simulink model "SensorlessHandover"  (R2026b)
settings: Solver=VariableStepAuto
undefined symbols (not defined in the file or in its folder): fusionCfg, handoverCfg
settings Model: Creator=24322  LastModifiedBy=24322

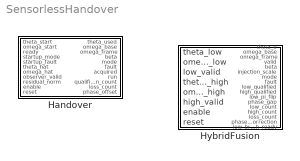
== system SensorlessHandover ==
  Handover : Subsystem  mask{handoverCfg=handoverCfg}
      mask prompts: handoverCfg "Handover configuration"
  HybridFusion : Subsystem  mask{fusionCfg=fusionCfg}
      mask prompts: fusionCfg "Two-tracker fusion configuration"

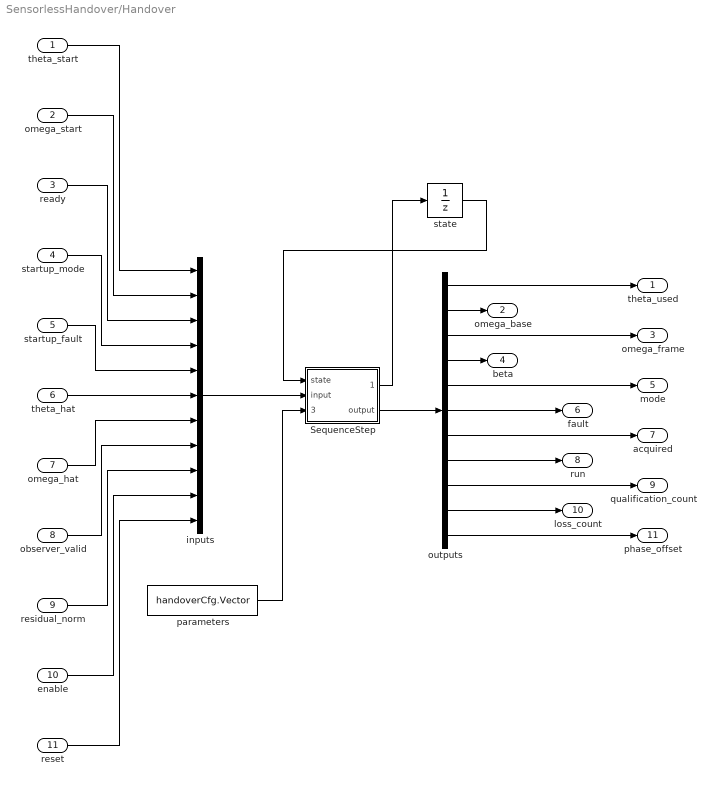
== system SensorlessHandover/Handover ==
  theta_start : Inport  SampleTime=handoverCfg.Ts
  omega_start : Inport  Port=2  SampleTime=handoverCfg.Ts
  ready : Inport  Port=3  SampleTime=handoverCfg.Ts
  startup_mode : Inport  Port=4  SampleTime=handoverCfg.Ts
  startup_fault : Inport  Port=5  SampleTime=handoverCfg.Ts
  theta_hat : Inport  Port=6  SampleTime=handoverCfg.Ts
  omega_hat : Inport  Port=7  SampleTime=handoverCfg.Ts
  observer_valid : Inport  Port=8  SampleTime=handoverCfg.Ts
  residual_norm : Inport  Port=9  SampleTime=handoverCfg.Ts
  enable : Inport  Port=10  SampleTime=handoverCfg.Ts
  reset : Inport  Port=11  SampleTime=handoverCfg.Ts
  SequenceStep : MATLAB Function  TreatAsAtomicUnit=on
  inputs : Mux  Inputs=11
  outputs : Demux  Outputs=11
  parameters : Constant  Value=handoverCfg.Vector
  state : UnitDelay  InitialCondition=handoverCfg.State0  SampleTime=handoverCfg.Ts
  theta_used : Outport
  omega_base : Outport  Port=2
  omega_frame : Outport  Port=3
  beta : Outport  Port=4
  mode : Outport  Port=5
  fault : Outport  Port=6
  acquired : Outport  Port=7
  run : Outport  Port=8
  qualification_count : Outport  Port=9
  loss_count : Outport  Port=10
  phase_offset : Outport  Port=11
  wires:
  outputs/11 -> phase_offset/1
  outputs/10 -> loss_count/1
  outputs/9 -> qualification_count/1
  outputs/8 -> run/1
  outputs/7 -> acquired/1
  outputs/6 -> fault/1
  outputs/5 -> mode/1
  outputs/4 -> beta/1
  outputs/3 -> omega_frame/1
  outputs/2 -> omega_base/1
  outputs/1 -> theta_used/1
  reset/1 -> inputs/11
  enable/1 -> inputs/10
  residual_norm/1 -> inputs/9
  observer_valid/1 -> inputs/8
  omega_hat/1 -> inputs/7
  theta_hat/1 -> inputs/6
  startup_fault/1 -> inputs/5
  startup_mode/1 -> inputs/4
  ready/1 -> inputs/3
  omega_start/1 -> inputs/2
  theta_start/1 -> inputs/1
  SequenceStep/2(output) -> outputs/1
  SequenceStep/1(nextState) -> state/1
  parameters/1 -> SequenceStep/3(parameter)
  inputs/1 -> SequenceStep/2(input)
  state/1 -> SequenceStep/1(state)

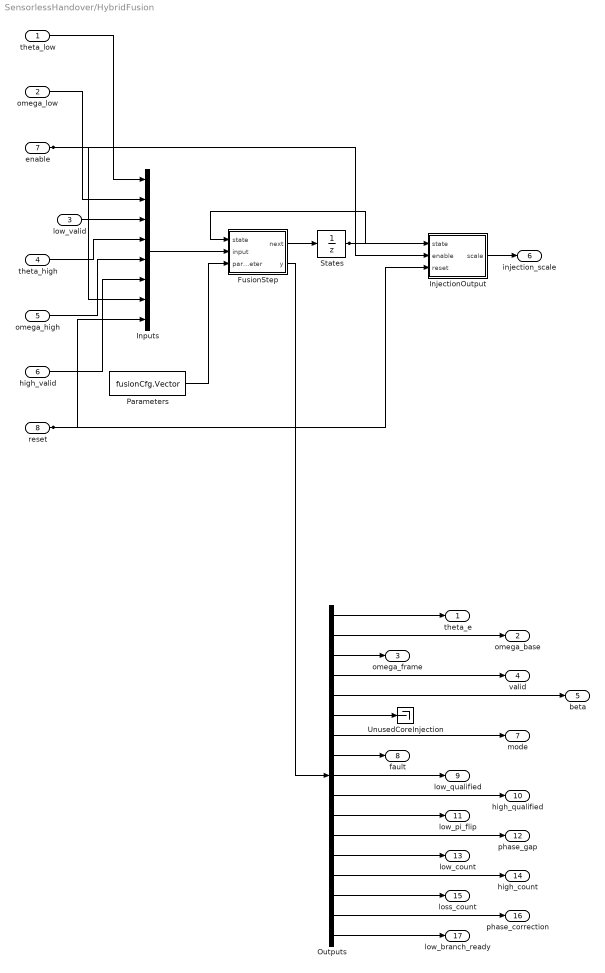
== system SensorlessHandover/HybridFusion ==
  theta_low : Inport  SampleTime=fusionCfg.Ts
  omega_low : Inport  Port=2  SampleTime=fusionCfg.Ts
  low_valid : Inport  Port=3  SampleTime=fusionCfg.Ts
  theta_high : Inport  Port=4  SampleTime=fusionCfg.Ts
  omega_high : Inport  Port=5  SampleTime=fusionCfg.Ts
  high_valid : Inport  Port=6  SampleTime=fusionCfg.Ts
  enable : Inport  Port=7  SampleTime=fusionCfg.Ts
  reset : Inport  Port=8  SampleTime=fusionCfg.Ts
  FusionStep : MATLAB Function  TreatAsAtomicUnit=on
  InjectionOutput : MATLAB Function  TreatAsAtomicUnit=on
  Inputs : Mux  Inputs=8
  Outputs : Demux  Outputs=17
  Parameters : Constant  Value=fusionCfg.Vector
  States : UnitDelay  InitialCondition=fusionCfg.State0  SampleTime=fusionCfg.Ts
  UnusedCoreInjection : Terminator
  theta_e : Outport
  omega_base : Outport  Port=2
  omega_frame : Outport  Port=3
  valid : Outport  Port=4
  beta : Outport  Port=5
  injection_scale : Outport  Port=6
  mode : Outport  Port=7
  fault : Outport  Port=8
  low_qualified : Outport  Port=9
  high_qualified : Outport  Port=10
  low_pi_flip : Outport  Port=11
  phase_gap : Outport  Port=12
  low_count : Outport  Port=13
  high_count : Outport  Port=14
  loss_count : Outport  Port=15
  phase_correction : Outport  Port=16
  low_branch_ready : Outport  Port=17
  wires:
  Outputs/17 -> low_branch_ready/1
  Outputs/16 -> phase_correction/1
  Outputs/15 -> loss_count/1
  Outputs/14 -> high_count/1
  Outputs/13 -> low_count/1
  Outputs/12 -> phase_gap/1
  Outputs/11 -> low_pi_flip/1
  Outputs/10 -> high_qualified/1
  Outputs/9 -> low_qualified/1
  Outputs/8 -> fault/1
  Outputs/7 -> mode/1
  InjectionOutput/1(scale) -> injection_scale/1
  Outputs/5 -> beta/1
  Outputs/4 -> valid/1
  Outputs/3 -> omega_frame/1
  Outputs/2 -> omega_base/1
  Outputs/1 -> theta_e/1
  reset/1 -> InjectionOutput/3(reset), Inputs/8
  enable/1 -> Inputs/7, InjectionOutput/2(enable)
  high_valid/1 -> Inputs/6
  omega_high/1 -> Inputs/5
  theta_high/1 -> Inputs/4
  low_valid/1 -> Inputs/3
  omega_low/1 -> Inputs/2
  theta_low/1 -> Inputs/1
  Outputs/6 -> UnusedCoreInjection/1
  FusionStep/2(y) -> Outputs/1
  FusionStep/1(next) -> States/1
  Parameters/1 -> FusionStep/3(parameter)
  Inputs/1 -> FusionStep/2(input)
  States/1 -> FusionStep/1(state), InjectionOutput/1(state)

== matlab function SensorlessHandover/HybridFusion/FusionStep ==
  data: next output; state input; y output; input input; parameter input
function [next,y]=hybrid_fusion_step(state,input,parameter)
%HYBRID_FUSION_STEP Qualified bidirectional fusion; no motor truth inputs.
% input: thetaLow,omegaLow,lowValid,thetaHigh,omegaHigh,highValid,enable,reset.
% y: theta,omegaBase,omegaFrame,valid,beta,injection,mode,fault,lowQ,highQ,
%    lowPiFlip,phaseGap,lowN,highN,lossN,phaseCorrection,lowBranchReady.
% Modes: 0 wait,1 low,2 blend,3 high,4 latched fault.
%#codegen
p=cast(parameter,'like',state);u=cast(input,'like',state);
next=state;y=zeros(17,1,'like',state);
if ~isfinite(u(7)) || ~isfinite(u(8))
    next(10)=2;next(4)=0;y(1)=state(1);y(7)=4;y(8)=2;return
end
if u(7)<.5 || u(8)>.5
    next(:)=0;next(4)=1;next(18)=1;return
end
if state(10)>0
    next(4)=0;y(1)=state(1);y(7)=4;y(8)=state(10);return
end

rawLow=all(isfinite(u(1:3))) && u(3)>.5 && abs(u(2))<=p(4) && state(4)>=p(17);
rawHigh=all(isfinite(u(4:6))) && u(6)>.5 && abs(u(5))>=p(16);
if rawLow && state(15)>.5
    rawLow=abs(wrap(u(1)-state(11)-p(1)*state(12)))<=p(14);
end
if rawHigh && state(16)>.5
    rawHigh=abs(wrap(u(4)-state(13)-p(1)*state(14)))<=p(14);
end
if rawLow
    next(11)=u(1);next(12)=u(2);next(15)=1;
elseif state(15)>.5
    next(11)=wrap(state(11)+p(1)*state(12));
end
if rawHigh
    next(13)=u(4);next(14)=u(5);next(16)=1;
elseif state(16)>.5
    next(13)=wrap(state(13)+p(1)*state(14));
end

flip=state(5);branch=state(17);gap=cast(0,'like',state);
if state(4)<p(17),branch=cast(0,'like',state);end
highWasQualified=state(7)>=p(7) && rawHigh;
if state(9)>.5 && state(3)>=1 && highWasQualified && rawLow && (branch<.5 || state(6)<1)
    ordinary=abs(wrap(u(1)-u(4)));opposite=abs(wrap(u(1)+pi-u(4)));
    candidate=cast(opposite<ordinary,'like',state);
    candidateGap=wrap(u(4)-u(1)-pi*candidate);
    if abs(candidateGap)<=p(5) && abs(u(2)-u(5))<=p(6)
        flip=candidate;branch=cast(1,'like',state);
    else
        branch=cast(0,'like',state);
    end
end
thetaLow=cast(0,'like',state);
if rawLow,thetaLow=wrap(u(1)+pi*flip);end
agree=false;
if rawLow && rawHigh
    gap=wrap(u(4)-thetaLow);
    agree=abs(gap)<=p(5) && abs(u(2)-u(5))<=p(6);
end
lowEligible=rawLow && (state(9)<.5 || branch>.5);
if state(9)>.5 && state(3)>0 && rawHigh,lowEligible=lowEligible && agree;end
highEligible=rawHigh;
if state(6)>=p(7) && rawLow,highEligible=highEligible && agree;end
if lowEligible
    next(6)=min(state(6)+1,p(7));next(19)=0;
else
    next(19)=min(state(19)+1,p(8));
    if state(6)<p(7) || next(19)>=p(8),next(6)=0;end
    if ~rawLow && next(19)>=p(8),next(15)=0;end
end
if highEligible
    next(7)=min(state(7)+1,p(7));next(20)=0;
else
    next(20)=min(state(20)+1,p(8));
    if state(7)<p(7) || next(20)>=p(8),next(7)=0;end
    if ~rawHigh && next(20)>=p(8),next(16)=0;end
end
lowQ=lowEligible && next(6)>=p(7);highQ=highEligible && next(7)>=p(7);
next(5)=flip;next(17)=branch;

beta=state(3);omega=state(2);theta=state(1);frameOmega=omega;correction=cast(0,'like',state);
valid=false;mode=cast(0,'like',state);fault=cast(0,'like',state);
if state(9)<.5
    if lowQ
        next(9)=1;branch=cast(1,'like',state);next(17)=branch;
        beta=cast(0,'like',state);theta=thetaLow;omega=u(2);frameOmega=omega;valid=true;
    elseif highQ && p(15)>.5 && abs(u(5))>=p(3)
        next(9)=1;beta=cast(1,'like',state);theta=wrap(u(4));omega=u(5);frameOmega=omega;valid=true;
    end
else
    available=lowQ || highQ;
    if available
        next(8)=0;
        if lowQ && highQ
            speed=abs((1-beta)*u(2)+beta*u(5));
            target=min(max((speed-p(2))/(p(3)-p(2)),0),1);
            beta=beta+min(max(target-beta,-p(9)),p(9));
            omega=(1-beta)*u(2)+beta*u(5);
            rawTheta=wrap(thetaLow+beta*gap);
        elseif lowQ
            beta=cast(0,'like',state);omega=u(2);rawTheta=thetaLow;
        else
            beta=cast(1,'like',state);omega=u(5);rawTheta=wrap(u(4));
        end
        prediction=wrap(state(1)+p(1)*omega);
        error=wrap(rawTheta-prediction);
        correction=min(max(error,-p(13)*p(1)),p(13)*p(1));
        theta=wrap(prediction+correction);
        frameOmega=wrap(theta-state(1))/p(1);valid=true;
    else
        next(8)=state(8)+1;
        theta=wrap(state(1)+p(1)*omega);frameOmega=omega;
        valid=next(8)<p(8);
        if ~valid,next(10)=1;fault=cast(1,'like',state);end
    end
end

if fault>0
    valid=false;mode=cast(4,'like',state);next(4)=0;next(18)=1;
elseif next(9)>.5
    if beta<=0,mode=cast(1,'like',state);
    elseif beta>=1,mode=cast(3,'like',state);
    else,mode=cast(2,'like',state);end
end
injectionTarget=state(18);
if next(9)<.5 || ~highQ || abs(omega)<=p(11)
    injectionTarget=cast(1,'like',state);
elseif beta>=1 && abs(omega)>=p(12)
    injectionTarget=cast(0,'like',state);
end
if fault==0
    next(4)=min(max(state(4)+min(max(injectionTarget-state(4),-p(10)),p(10)),0),1);
end
next(18)=injectionTarget;next(1)=theta;next(2)=omega;next(3)=beta;
y(1)=theta;y(2)=omega;y(3)=frameOmega;y(4)=cast(valid,'like',state);y(5)=beta;
y(6)=state(4);y(7)=mode;y(8)=fault;y(9)=cast(lowQ,'like',state);y(10)=cast(highQ,'like',state);
y(11)=flip;y(12)=gap;y(13)=next(6);y(14)=next(7);y(15)=next(8);y(16)=correction;y(17)=branch;
end
function angle=wrap(angle)
angle=atan2(sin(angle),cos(angle));
end

== matlab function SensorlessHandover/Handover/SequenceStep ==
  data: state input; nextState output; input input; parameter input; output output
function [nextState,output]=handover_step(state,input,parameter)
%#codegen
%HANDOVER_STEP Unit Delay owns all states; no plant truth is an input.
% input: thetaStart,omegaStart,ready,startMode,startFault,thetaHat,omegaHat,
%        observerValid,currentResidualNorm,enable,reset.
% output: thetaUsed,omegaBase,omegaFrame,beta,mode,fault,acquired,run,
%         qualificationN,lossN,phaseOffset.
p=cast(parameter,'like',state);u=cast(input,'like',state);
nextState=state;output=zeros(11,1,'like',state);
thetaStart=u(1);thetaHat=u(6);omegaHat=u(7);mode=state(1);
if u(10)<0.5 || u(11)>0.5
    nextState(:)=0;nextState(6)=thetaStart;output(1)=thetaStart;
    return
end
fraction=min(state(3)/p(7),1);beta=fraction*fraction*(3-2*fraction);offset=state(5);
if mode==5
    output(1)=state(6);output(4)=beta;output(5)=5;output(6)=state(7);
    output(9)=state(2);output(10)=state(4);output(11)=offset;
    return
end
if mode<=2 && u(5)>0.5
    nextState(1)=5;nextState(7)=1;
    output(1)=state(6);output(5)=5;output(6)=1;
    output(9)=state(2);output(10)=state(4);output(11)=offset;
    return
end
theta=thetaStart;omegaBase=u(2);omegaFrame=omegaBase;
baseHealthy=u(8)>0.5 && abs(omegaHat)>=p(2) && u(9)>=0 && u(9)<=p(5);
if mode==0
    nextState(1)=1;nextState(2)=0;
    nextState(8)=thetaHat;nextState(9)=omegaHat;
elseif mode==1 || mode==2
    phaseGap=atan2(sin(thetaStart-thetaHat),cos(thetaStart-thetaHat));
    ordinary=u(3)>0.5 && abs(u(2)-omegaHat)<=p(3) && abs(phaseGap)<=p(4);
    flying=p(10)>0.5 && u(4)==1;
    if baseHealthy && (ordinary || flying)
        nextState(1)=2;nextState(2)=min(state(2)+1,p(6));
        if nextState(2)>=p(6)
            nextState(1)=3;nextState(3)=0;nextState(4)=0;nextState(5)=phaseGap;
        end
    else
        nextState(1)=1;nextState(2)=0;
    end
    nextState(8)=thetaHat;nextState(9)=omegaHat;
elseif mode==3 || mode==4
    prediction=state(8)+p(1)*state(9);
    prediction=atan2(sin(prediction),cos(prediction));
    innovation=atan2(sin(thetaHat-prediction),cos(thetaHat-prediction));
    healthy=baseHealthy && abs(innovation)<=p(9);
    if healthy
        safeTheta=thetaHat;safeOmega=omegaHat;nextState(4)=0;
    else
        safeTheta=prediction;safeOmega=state(9);nextState(4)=state(4)+1;
    end
    nextState(8)=safeTheta;nextState(9)=safeOmega;
    if mode==3 && state(3)==0
        offset=atan2(sin(thetaStart-safeTheta),cos(thetaStart-safeTheta));
        nextState(5)=offset;
    end
    if mode==4,beta=cast(1,'like',state);end
    theta=safeTheta+(1-beta)*offset;theta=atan2(sin(theta),cos(theta));
    omegaBase=safeOmega;omegaFrame=safeOmega;
    if mode==3 && healthy
        if beta<1
            nextState(3)=min(state(3)+1,p(7));
            nextFraction=nextState(3)/p(7);
            nextBeta=nextFraction*nextFraction*(3-2*nextFraction);
            omegaFrame=safeOmega-offset*(nextBeta-beta)/p(1);
        else
            nextState(1)=4;
        end
    end
    if mode==3 && state(3)==0 && ~healthy,omegaFrame=u(2);end
    if nextState(4)>=p(8),nextState(1)=5;nextState(7)=2;end
else
    nextState(1)=5;nextState(7)=3;
    output(1)=state(6);output(5)=5;output(6)=3;
    return
end
nextState(6)=theta;
output(1)=theta;output(2)=omegaBase;output(3)=omegaFrame;output(4)=beta;
output(5)=mode;output(6)=state(7);output(7)=cast(mode==4,'like',state);
output(8)=cast(mode~=0,'like',state);output(9)=state(2);
output(10)=state(4);output(11)=offset;
end

== matlab function SensorlessHandover/HybridFusion/InjectionOutput ==
  data: state input; scale output; enable input; reset input
function scale=hybrid_injection_output(state,enable,reset)
%HYBRID_INJECTION_OUTPUT State-only scheduler avoids an observer algebraic loop.
%#codegen
scale=cast(0,'like',state);
if isfinite(enable) && isfinite(reset) && enable>.5 && reset<.5 && state(10)==0
    scale=state(4);
end
end
